simulink model "HorizontalEstimatorTest"  (R2026b)
settings: Solver=FixedStepDiscrete  StopTime=1  FixedStep=.0025
settings Model: Creator=tyasukaw  LastModifiedBy=tyasukaw

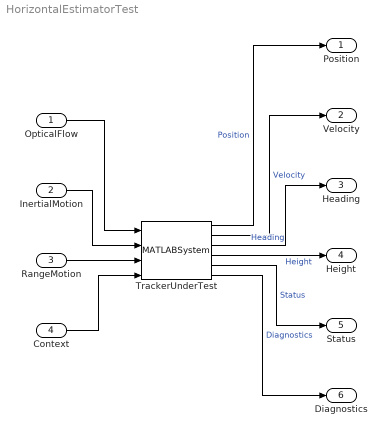
== system HorizontalEstimatorTest ==
  OpticalFlow : Inport  OutDataTypeStr=Bus: HorizontalFlowBus  SampleTime=.0025
  InertialMotion : Inport  Port=2  OutDataTypeStr=Bus: HorizontalInertialBus  SampleTime=.0025
  RangeMotion : Inport  Port=3  OutDataTypeStr=Bus: HorizontalRangeBus  SampleTime=.0025
  Context : Inport  Port=4  OutDataTypeStr=Bus: HorizontalContextBus  SampleTime=.0025
  TrackerUnderTest : MATLABSystem  System=horizontal.FlowMotion  SampleTime=.0025  WindowSamples=8  XCountsPerRad=385  YCountsPerRad=385  MinQuality=25  MinHeightM=.12  MaxHeightM=1.0  MaxRangeAgeS=.15  MaxFlowAgeS=.025  MaxSampleGapS=.01  MaxSpeedMps=1.5  MaxVerticalSpeedMps=2.0  MaxTiltDeg=25  VelocityTimeConstantS=.05  SimulateUsing=Code generation
      mask Type: horizontal.FlowMotion
  Position : Outport
  Velocity : Outport  Port=2
  Heading : Outport  Port=3
  Height : Outport  Port=4
  Status : Outport  Port=5
  Diagnostics : Outport  Port=6
  wires:
  TrackerUnderTest/6 -> Diagnostics/1  "Diagnostics"
  TrackerUnderTest/5 -> Status/1  "Status"
  TrackerUnderTest/4 -> Height/1  "Height"
  TrackerUnderTest/3 -> Heading/1  "Heading"
  TrackerUnderTest/2 -> Velocity/1  "Velocity"
  TrackerUnderTest/1 -> Position/1  "Position"
  Context/1 -> TrackerUnderTest/4
  RangeMotion/1 -> TrackerUnderTest/3
  InertialMotion/1 -> TrackerUnderTest/2
  OpticalFlow/1 -> TrackerUnderTest/1
